simulink model "SensorlessIF"  (R2026b)
settings: Solver=FixedStepDiscrete  StopTime=experimentCfg.Duration  FixedStep=experimentCfg.Step
PostLoadFcn:
  | addpath(fullfile(fileparts(get_param(bdroot,'FileName')),'..','build_process'));initialize_if_app(bdroot);
model workspace (MAT data in the model file):
  bridgeCfg.Rs = 0.5
  bridgeCfg.Ld = 0.001
  bridgeCfg.Lq = 0.001
  bridgeCfg.Flux = 0.035
  bridgeCfg.PolePairs = 4
  bridgeCfg.J = 0.0005
  bridgeCfg.B = 0.001
  bridgeCfg.Id0 = 0
  bridgeCfg.Iq0 = 0
  bridgeCfg.Speed0 = 0
  bridgeCfg.Position0 = 0
  bridgeCfg.Ts = 1.25e-05
  bridgeCfg.Vdc = 48
  bridgeCfg.DiodeVf = 0.7
  bridgeCfg.DiodeRon = 0.01
  bridgeCfg.MechanicalEnabled = 1
  bridgeCfg.CurrentTolerance = 1e-09
  bridgeCfg.VoltageTolerance = 1e-08
  bridgeCfg.MaxCurrent = 200
  bridgeCfg.MaxSpeed = 1000
  bridgeCfg.MaxAngleStep = 0.1
  bridgeCfg.State0 = [0; 0; 0; 0]
  bridgeCfg.Vector = [1.25e-05; 0.5; 0.001; 0.001; 0.035; 4; 0.0005; 0.001; 48; 0.7; 0.01; 1; 1e-09; 1e-08; 200; 1000; 0.1]
  currentCfg.Ts = 6.25e-05
  currentCfg.BandwidthHz = 500
  currentCfg.Kpd = 3.14159265359
  currentCfg.Kpq = 3.14159265359
  currentCfg.Kid = 1570.79632679
  currentCfg.Kiq = 1570.79632679
  currentCfg.Kaw = 16000
  experimentCfg.Duration = 2
  experimentCfg.Step = 1.25e-05
  experimentCfg.Frequency = 40
  experimentCfg.LoadTorque = 0.05
  experimentCfg.LoadTime = 1.5
  experimentCfg.LogPeriod = 0.001
  inverterCfg.Vdc = 1
  inverterCfg.MinDuty = 0.02
  inverterCfg.PwmTs = 6.25e-05
  inverterCfg.LinearLimit = 0.554256258422
  motorCfg.Rs = 0.5
  motorCfg.Ld = 0.001
  motorCfg.Lq = 0.001
  motorCfg.Flux = 0.035
  motorCfg.PolePairs = 4
  motorCfg.J = 0.0005
  motorCfg.B = 0.001
  motorCfg.Id0 = 0
  motorCfg.Iq0 = 0
  motorCfg.Speed0 = 0
  motorCfg.Position0 = 0
  openLoopCfg.Ts = 6.25e-05
  openLoopCfg.Kind = 1
  openLoopCfg.MaximumFrequency = 80
  openLoopCfg.FrequencySlew = 40
  openLoopCfg.ObserveTime = 0.05
  openLoopCfg.StartVoltageMaximum = 0.25
  openLoopCfg.StartCurrentMaximum = 0.2
  openLoopCfg.ObserveTimeout = 0.5
  openLoopCfg.AlignTime = 0.25
  openLoopCfg.AlignRampTime = 0.1
  openLoopCfg.AlignAmplitude = 2
  openLoopCfg.RunAmplitude = 3
  openLoopCfg.AmplitudeSlew = 40
  openLoopCfg.VfSlope = 0.219911485751
  openLoopCfg.VfBoost = 0.5
  openLoopCfg.VoltageFraction = 0.554256258422
  openLoopCfg.CurrentTrip = 12
  openLoopCfg.Theta0 = 0
  openLoopCfg.ObserveTicks = 800
  openLoopCfg.ObserveTimeoutTicks = 8000
  openLoopCfg.AlignTicks = 4000
  openLoopCfg.AlignRampTicks = 1600
  openLoopCfg.Vector = [6.25e-05; 1; 80; 40; 800; 0.25; 0.2; 8000; 4000; 1600; 2; 3; 40; 0.219911485751; 0.5; 0.554256258422; 12; 0]
  openLoopCfg.State0 = [0; 0; 0; 0; 0; 0; 0; 0]
  powerCfg.Vdc = 48
  powerCfg.MinDuty = 0.02
  testStim.time = []
  testStim.signals.values = [40 40 40 40 40 40 40 40 40 40 40 40 ... (160005 elements, 32001x5)]
  testStim.signals.dimensions = 5
libraries: CurrentControl x2, ClarkePark x2, OpenLoopDrive x1, PMSMBridgeBusPlant x1, Inverter x1
settings Model: Creator=24322  LastModifiedBy=24322

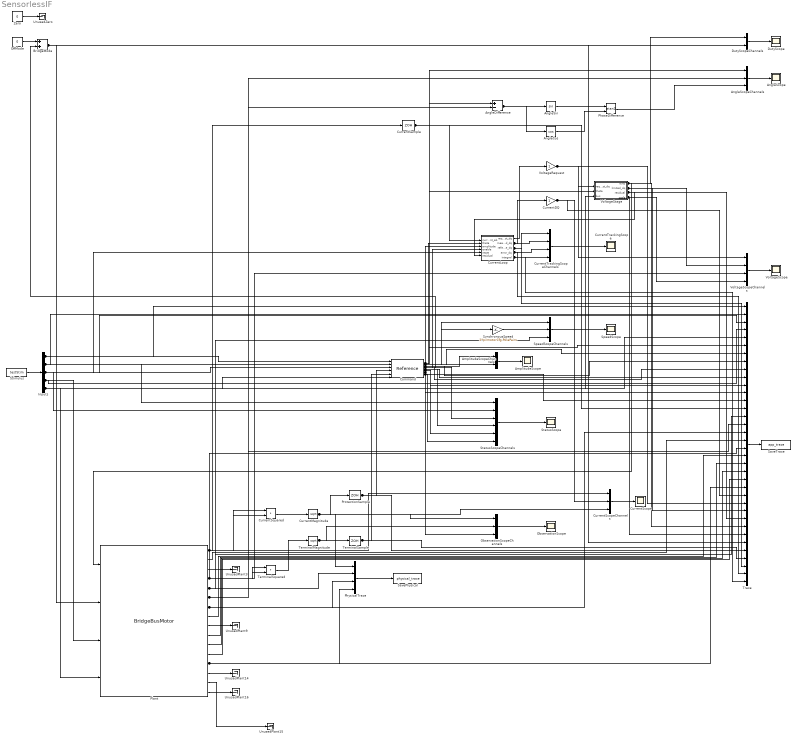
== system SensorlessIF ==
  AmplitudeScope : Scope
  AmplitudeScopeChannels : Mux  Inputs=2
  AngleCos : Trigonometry  Operator=cos
  AngleDifference : Sum  Inputs=+-
  AngleScope : Scope
  AngleScopeChannels : Mux  Inputs=3
  AngleSin : Trigonometry
  BridgeMode : Sum
  Command : OpenLoopDrive/Reference  openLoopCfg=openLoopCfg
  CurrentDQ : Gain
  CurrentLoop : Subsystem
  CurrentMagnitude : Sqrt
  CurrentSample : ZeroOrderHold  SampleTime=currentCfg.Ts
  CurrentScope : Scope
  CurrentScopeChannels : Mux  Inputs=3
  CurrentSquared : DotProduct  OutDataTypeStr=Inherit: Inherit via internal rule
  CurrentTrackingScope : Scope
  CurrentTrackingScopeChannels : Mux
  DutyScope : Scope
  DutyScopeChannels : Mux  Inputs=2
  Inputs : Demux  Outputs=5
  ObservationScope : Scope
  ObservationScopeChannels : Mux  Inputs=3
  OffMode : Constant  Value=0
  PhaseDifference : Trigonometry  Operator=atan2
  PhysicalTrace : Mux
  Plant : PMSMBridgeBusPlant/BridgeBusMotor  cfg=bridgeCfg
  ProtectionSample : ZeroOrderHold  SampleTime=currentCfg.Ts
  SavePhysical : ToWorkspace  VariableName=physical_trace  SaveFormat=Structure With Time  SampleTime=bridgeCfg.Ts
  SaveTrace : ToWorkspace  VariableName=app_trace  SaveFormat=Structure With Time  SampleTime=currentCfg.Ts
  SpeedScope : Scope
  SpeedScopeChannels : Mux  Inputs=3
  StatusScope : Scope
  StatusScopeChannels : Mux  Inputs=6
  Stimulus : FromWorkspace  VariableName=testStim  SampleTime=currentCfg.Ts  Interpolate=off  OutputAfterFinalValue=Holding final value
  SynchronousSpeed : Gain  Gain=2*pi/motorCfg.PolePairs
  TerminalMagnitude : Sqrt
  TerminalSample : ZeroOrderHold  SampleTime=currentCfg.Ts
  TerminalSquared : DotProduct  OutDataTypeStr=Inherit: Inherit via internal rule
  Trace : Mux  Inputs=36
  UnusedPlant{3,9,14..16} (5 alike) : Terminator
  UnusedZero : Terminator
  VoltageRequest : Gain
  VoltageScope : Scope
  VoltageScopeChannels : Mux
  VoltageStage : Subsystem
  Zero : Constant  Value=0
  wires:
  Zero/1 -> UnusedZero/1
  CurrentTrackingScopeChannels/1 -> CurrentTrackingScope/1
  AmplitudeScopeChannels/1 -> AmplitudeScope/1
  ObservationScopeChannels/1 -> ObservationScope/1
  StatusScopeChannels/1 -> StatusScope/1
  DutyScopeChannels/1 -> DutyScope/1
  VoltageScopeChannels/1 -> VoltageScope/1
  CurrentScopeChannels/1 -> CurrentScope/1
  PhaseDifference/1 -> AngleScopeChannels/3
  AngleScopeChannels/1 -> AngleScope/1
  SynchronousSpeed/1 -> SpeedScopeChannels/2
  SpeedScopeChannels/1 -> SpeedScope/1
  CurrentLoop/5(integral) -> Trace/36, CurrentTrackingScopeChannels/4
  CurrentLoop/4(error_dq) -> Trace/35, CurrentTrackingScopeChannels/3
  CurrentLoop/3(reference_dq) -> Trace/34, CurrentTrackingScopeChannels/1
  VoltageStage/4(scale) -> Trace/30, VoltageScopeChannels/4
  VoltageStage/2(limited_dq) -> Trace/27, VoltageScopeChannels/2
  CurrentDQ/1 -> Trace/25, CurrentScopeChannels/2
  Plant/12 -> Trace/23
  Plant/11 -> Trace/22
  Plant/10 -> Trace/21
  Plant/8 -> Trace/20
  Plant/2 -> Trace/18
  Command/8 -> Trace/13, StatusScopeChannels/6
  Command/7 -> Trace/12, ObservationScopeChannels/3
  Command/6 -> Trace/11, StatusScopeChannels/5
  Command/5 -> Trace/10, StatusScopeChannels/4
  Plant/13 -> PhysicalTrace/4, Trace/24
  Plant/7 -> PhysicalTrace/3, Trace/17
  Plant/5 -> PhysicalTrace/2, Trace/15, SpeedScopeChannels/3
  AngleCos/1 -> PhaseDifference/2
  AngleSin/1 -> PhaseDifference/1
  AngleDifference/1 -> AngleSin/1, AngleCos/1
  Plant/6 -> AngleDifference/2, Trace/16, AngleScopeChannels/2
  Command/2 -> Trace/7, SpeedScopeChannels/1, SynchronousSpeed/1, AmplitudeScopeChannels/2
  PhysicalTrace/1 -> SavePhysical/1
  Trace/1 -> SaveTrace/1
  CurrentLoop/1(request_dq) -> VoltageRequest/1
  CurrentLoop/2(measured_dq) -> CurrentDQ/1, CurrentTrackingScopeChannels/2
  Inputs/1 -> Command/1, Trace/1
  Inputs/2 -> Command/2, Trace/2, StatusScopeChannels/1
  Inputs/3 -> CurrentLoop/5(reset), Command/3, Trace/3, StatusScopeChannels/2
  Inputs/5 -> VoltageStage/3(bus), Command/6, Plant/4, Trace/5
  CurrentMagnitude/1 -> ProtectionSample/1, CurrentScopeChannels/3, PhysicalTrace/1, ObservationScopeChannels/1
  ProtectionSample/1 -> Command/4, Trace/32
  TerminalMagnitude/1 -> ObservationScopeChannels/2, TerminalSample/1
  TerminalSample/1 -> Trace/33, Command/5
  Plant/1 -> CurrentSquared/2, CurrentSquared/1, CurrentSample/1, CurrentScopeChannels/1
  CurrentSquared/1 -> CurrentMagnitude/1
  Plant/4 -> TerminalSquared/1, TerminalSquared/2, Trace/19, VoltageScopeChannels/3
  TerminalSquared/1 -> TerminalMagnitude/1
  Stimulus/1 -> Inputs/1
  OffMode/1 -> BridgeMode/1
  Command/4 -> CurrentLoop/4(enable), BridgeMode/2, Trace/9, StatusScopeChannels/3
  BridgeMode/1 -> Plant/2, Trace/31, DutyScopeChannels/2
  Inputs/4 -> Plant/3, Trace/4
  VoltageStage/1(duty) -> Plant/1, Trace/29, DutyScopeChannels/1
  VoltageRequest/1 -> VoltageStage/1(request_dq), Trace/26, VoltageScopeChannels/1
  Command/1 -> CurrentLoop/2(theta), VoltageStage/2(theta), AngleDifference/1, Trace/6, AngleScopeChannels/1
  CurrentSample/1 -> Trace/14, CurrentLoop/1(current_ab)
  Command/3 -> CurrentLoop/3(amplitude), Trace/8, AmplitudeScopeChannels/1
  VoltageStage/3(residual) -> CurrentLoop/6(residual), Trace/28
  Plant/3 -> UnusedPlant3/1
  Plant/9 -> UnusedPlant9/1
  Plant/14 -> UnusedPlant14/1
  Plant/15 -> UnusedPlant15/1
  Plant/16 -> UnusedPlant16/1

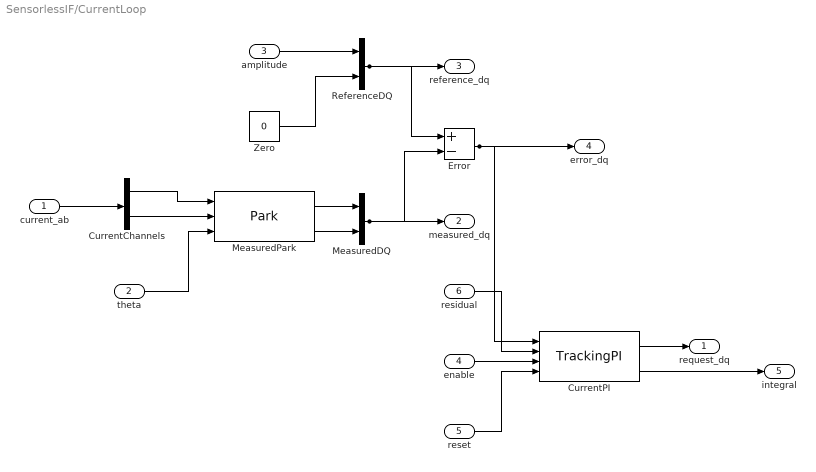
== system SensorlessIF/CurrentLoop ==
  current_ab : Inport
  theta : Inport  Port=2
  amplitude : Inport  Port=3
  enable : Inport  Port=4
  reset : Inport  Port=5
  residual : Inport  Port=6
  CurrentChannels : Demux  Outputs=2
  CurrentPI : CurrentControl/TrackingPI  SystemSampleTime=-1  VariantActivationTime=update diagram  EmptyChoice=off  PassThrough=off  PassThroughVariantControl=(default)  EmptyChoiceVariantControl=(default)  AllowFlexibleInterface=on  Latency=0  AutoFrameSizeCalculation=off
  Error : Sum  Inputs=+-
  MeasuredDQ : Mux  Inputs=2
  MeasuredPark : ClarkePark/Park  SystemSampleTime=-1  VariantActivationTime=update diagram  EmptyChoice=off  PassThrough=off  PassThroughVariantControl=(default)  EmptyChoiceVariantControl=(default)  AllowFlexibleInterface=on  Latency=0  AutoFrameSizeCalculation=off
  ReferenceDQ : Mux  Inputs=2
  Zero : Constant  Value=0
  request_dq : Outport
  measured_dq : Outport  Port=2
  reference_dq : Outport  Port=3
  error_dq : Outport  Port=4
  integral : Outport  Port=5
  wires:
  CurrentPI/2 -> integral/1
  CurrentPI/1 -> request_dq/1
  reset/1 -> CurrentPI/4
  enable/1 -> CurrentPI/3
  residual/1 -> CurrentPI/2
  Error/1 -> CurrentPI/1, error_dq/1
  MeasuredDQ/1 -> Error/2, measured_dq/1
  ReferenceDQ/1 -> Error/1, reference_dq/1
  Zero/1 -> ReferenceDQ/2
  amplitude/1 -> ReferenceDQ/1
  MeasuredPark/2 -> MeasuredDQ/2
  MeasuredPark/1 -> MeasuredDQ/1
  theta/1 -> MeasuredPark/3
  CurrentChannels/2 -> MeasuredPark/2
  CurrentChannels/1 -> MeasuredPark/1
  current_ab/1 -> CurrentChannels/1

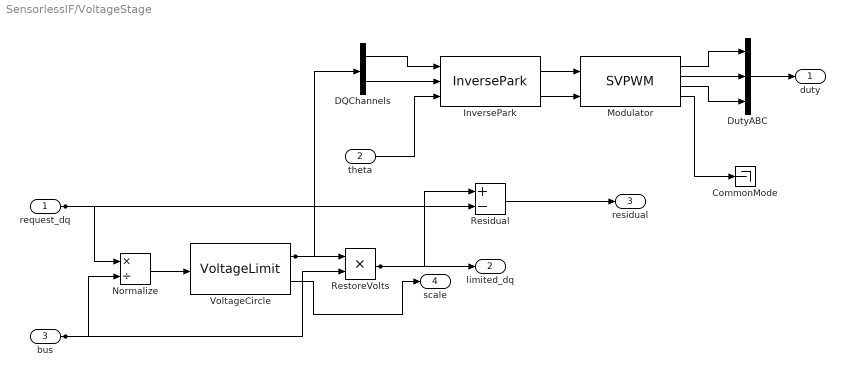
== system SensorlessIF/VoltageStage ==
  request_dq : Inport
  theta : Inport  Port=2
  bus : Inport  Port=3
  CommonMode : Terminator
  DQChannels : Demux  Outputs=2
  DutyABC : Mux  Inputs=3
  InversePark : ClarkePark/InversePark  SystemSampleTime=-1  VariantActivationTime=update diagram  EmptyChoice=off  PassThrough=off  PassThroughVariantControl=(default)  EmptyChoiceVariantControl=(default)  AllowFlexibleInterface=on  Latency=0  AutoFrameSizeCalculation=off
  Modulator : Inverter/SVPWM  SystemSampleTime=-1  VariantActivationTime=update diagram  EmptyChoice=off  PassThrough=off  PassThroughVariantControl=(default)  EmptyChoiceVariantControl=(default)  AllowFlexibleInterface=on  Latency=0  AutoFrameSizeCalculation=off
  Normalize : Product  Inputs=*/
  Residual : Sum  Inputs=+-
  RestoreVolts : Product  Inputs=**
  VoltageCircle : CurrentControl/VoltageLimit  SystemSampleTime=-1  VariantActivationTime=update diagram  EmptyChoice=off  PassThrough=off  PassThroughVariantControl=(default)  EmptyChoiceVariantControl=(default)  AllowFlexibleInterface=on  Latency=0  AutoFrameSizeCalculation=off
  duty : Outport
  limited_dq : Outport  Port=2
  residual : Outport  Port=3
  scale : Outport  Port=4
  wires:
  Modulator/3 -> DutyABC/3
  Modulator/2 -> DutyABC/2
  Modulator/1 -> DutyABC/1
  DutyABC/1 -> duty/1
  Modulator/4 -> CommonMode/1
  InversePark/2 -> Modulator/2
  InversePark/1 -> Modulator/1
  theta/1 -> InversePark/3
  DQChannels/2 -> InversePark/2
  DQChannels/1 -> InversePark/1
  VoltageCircle/2 -> scale/1
  Residual/1 -> residual/1
  RestoreVolts/1 -> limited_dq/1, Residual/1
  VoltageCircle/1 -> RestoreVolts/1, DQChannels/1
  Normalize/1 -> VoltageCircle/1
  bus/1 -> Normalize/2, RestoreVolts/2
  request_dq/1 -> Normalize/1, Residual/2
